simulink model "sf_aircraft_controller"  (R2025b)
settings: configuration reference "SharedConfig" (kept outside this file)
libraries: sf_aircraft_lib x4
settings Model: DataDictionary=sf_aircraft_dd.sldd  Creator=The MathWorks, Inc.  LastModifiedBy=The MathWorks, Inc.
settings ConfigSetRef: SourceName=SharedConfig

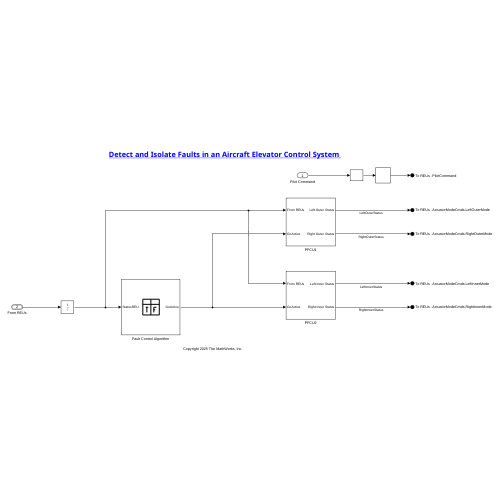
[thumbnail: Simulink's stored preview of the top-level diagram]
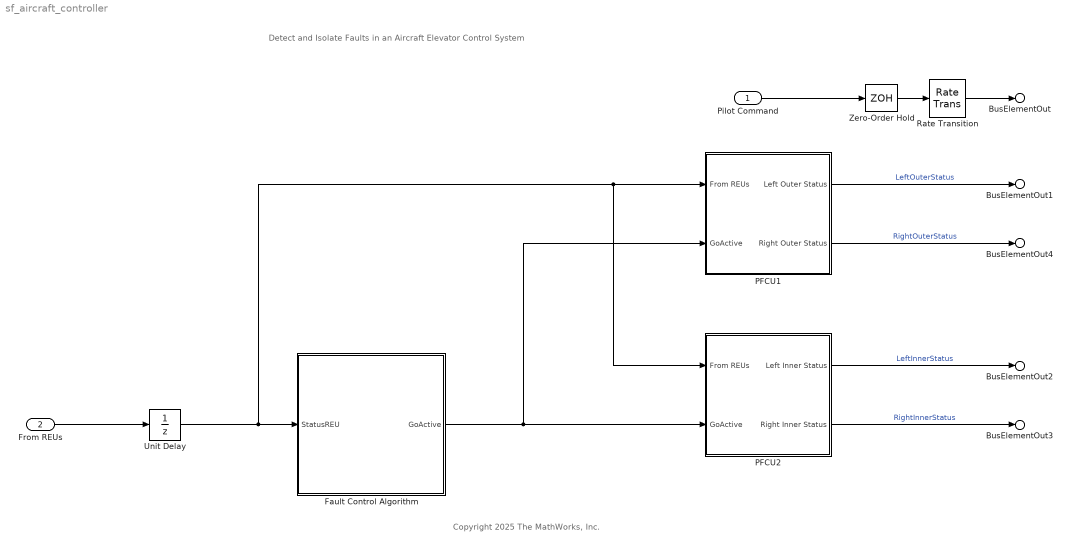
== system sf_aircraft_controller ==
  note: Copyright 2025 The MathWorks, Inc.
  note: Detect and Isolate Faults in an Aircraft Elevator Control System
  Pilot Command : Inport
  From REUs : Inport  Port=2  OutDataTypeStr=Bus: REUtoPFCU_type  PortDimensions=1  BusOutputAsStruct=on
  Fault Control Algorithm : Truth Table  TreatAsAtomicUnit=on
  PFCU1 : Subsystem
  PFCU2 : Subsystem
  Rate Transition : RateTransition  OutPortSampleTime=.01
  Unit Delay : UnitDelay  SampleTime=-1  HasFrameUpgradeWarning=on
  Zero-Order Hold : ZeroOrderHold  SampleTime=.1
  BusElementOut1 : Outport  PortName=To REUs  Element=ActuatorModeCmds.LeftOuterMode
  BusElementOut2 : Outport  PortName=To REUs  Element=ActuatorModeCmds.LeftInnerMode
  BusElementOut3 : Outport  PortName=To REUs  Element=ActuatorModeCmds.RightInnerMode
  BusElementOut4 : Outport  PortName=To REUs  Element=ActuatorModeCmds.RightOuterMode
  BusElementOut : Outport  PortName=To REUs  Element=PilotCommand
  wires:
  From REUs/1 -> Unit Delay/1
  Fault Control Algorithm/1(GoActive) -> PFCU1/2(GoActive), PFCU2/2(GoActive)
  Pilot Command/1 -> Zero-Order Hold/1
  PFCU1/1(Left Outer Status) -> BusElementOut1/1  "LeftOuterStatus"
  PFCU2/1(Left Inner Status) -> BusElementOut2/1  "LeftInnerStatus"
  PFCU2/2(Right Inner Status) -> BusElementOut3/1  "RightInnerStatus"
  PFCU1/2(Right Outer Status) -> BusElementOut4/1  "RightOuterStatus"
  Zero-Order Hold/1 -> Rate Transition/1
  Rate Transition/1 -> BusElementOut/1
  Unit Delay/1 -> PFCU1/1(From REUs), PFCU2/1(From REUs), Fault Control Algorithm/1(StatusREU)

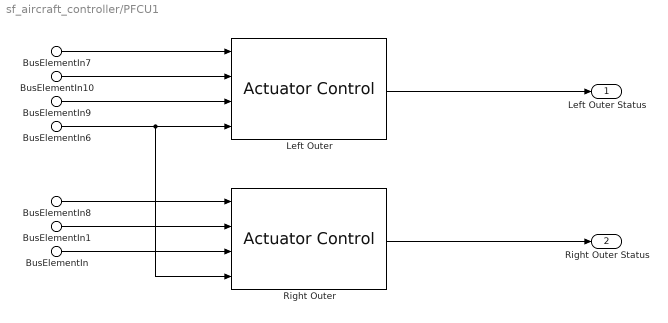
== system sf_aircraft_controller/PFCU1 ==
  BusElementIn6 : Inport  PortName=From REUs  Element=ResetCmd
  BusElementIn : Inport  PortName=From REUs  Element=RightOuterREUout.PositionFailureStatus
  BusElementIn1 : Inport  PortName=From REUs  Element=RightOuterREUout.HydraulicFailureStatus
  BusElementIn9 : Inport  PortName=From REUs  Element=LeftOuterREUout.PositionFailureStatus
  BusElementIn10 : Inport  PortName=From REUs  Element=LeftOuterREUout.HydraulicFailureStatus
  BusElementIn7 : Inport  Port=2  PortName=GoActive  Element=LeftOuterCmd
  BusElementIn8 : Inport  Port=2  PortName=GoActive  Element=RightOuterCmd
  Left Outer : sf_aircraft_lib/Actuator Control  SystemSampleTime=-1  VariantActivationTime=update diagram  EmptyChoice=off  PassThrough=off  PassThroughVariantControl=(default)  EmptyChoiceVariantControl=(default)  AllowFlexibleInterface=on  Latency=0  AutoFrameSizeCalculation=off
  Right Outer : sf_aircraft_lib/Actuator Control  SystemSampleTime=-1  VariantActivationTime=update diagram  EmptyChoice=off  PassThrough=off  PassThroughVariantControl=(default)  EmptyChoiceVariantControl=(default)  AllowFlexibleInterface=on  Latency=0  AutoFrameSizeCalculation=off
  Left Outer Status : Outport
  Right Outer Status : Outport  Port=2
  wires:
  Left Outer/1 -> Left Outer Status/1
  BusElementIn9/1 -> Left Outer/3
  BusElementIn10/1 -> Left Outer/2
  BusElementIn7/1 -> Left Outer/1
  Right Outer/1 -> Right Outer Status/1
  BusElementIn8/1 -> Right Outer/1
  BusElementIn1/1 -> Right Outer/2
  BusElementIn/1 -> Right Outer/3
  BusElementIn6/1 -> Right Outer/4, Left Outer/4

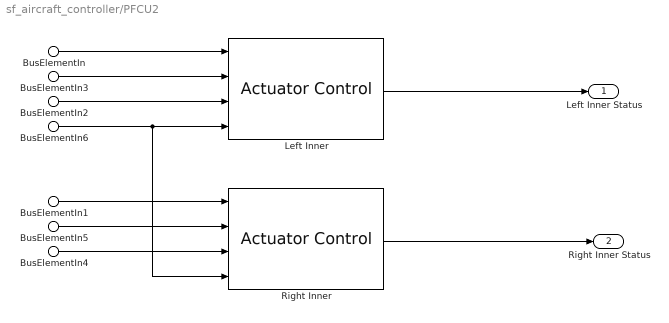
== system sf_aircraft_controller/PFCU2 ==
  BusElementIn2 : Inport  PortName=From REUs  Element=LeftInnerREUout.PositionFailureStatus
  BusElementIn3 : Inport  PortName=From REUs  Element=LeftInnerREUout.HydraulicFailureStatus
  BusElementIn4 : Inport  PortName=From REUs  Element=RightInnerREUout.PositionFailureStatus
  BusElementIn5 : Inport  PortName=From REUs  Element=RightInnerREUout.HydraulicFailureStatus
  BusElementIn6 : Inport  PortName=From REUs  Element=ResetCmd
  BusElementIn : Inport  Port=2  PortName=GoActive  Element=LeftInnerCmd
  BusElementIn1 : Inport  Port=2  PortName=GoActive  Element=RightInnerCmd
  Left Inner : sf_aircraft_lib/Actuator Control  SystemSampleTime=-1  VariantActivationTime=update diagram  EmptyChoice=off  PassThrough=off  PassThroughVariantControl=(default)  EmptyChoiceVariantControl=(default)  AllowFlexibleInterface=on  Latency=0  AutoFrameSizeCalculation=off
  Right Inner : sf_aircraft_lib/Actuator Control  SystemSampleTime=-1  VariantActivationTime=update diagram  EmptyChoice=off  PassThrough=off  PassThroughVariantControl=(default)  EmptyChoiceVariantControl=(default)  AllowFlexibleInterface=on  Latency=0  AutoFrameSizeCalculation=off
  Left Inner Status : Outport
  Right Inner Status : Outport  Port=2
  wires:
  Left Inner/1 -> Left Inner Status/1
  BusElementIn2/1 -> Left Inner/3
  BusElementIn3/1 -> Left Inner/2
  BusElementIn/1 -> Left Inner/1
  Right Inner/1 -> Right Inner Status/1
  BusElementIn1/1 -> Right Inner/1
  BusElementIn5/1 -> Right Inner/2
  BusElementIn4/1 -> Right Inner/3
  BusElementIn6/1 -> Right Inner/4, Left Inner/4

== matlab function sf_aircraft_controller/Fault Control Algorithm ==
  data: StatusREU input Bus: REUtoPFCU_type size=1; GoActive output Bus: PFCC_type
function GoActive = fcn(StatusREU)

aVarTruthTableCondition_1 = false;
aVarTruthTableCondition_2 = false;
aVarTruthTableCondition_3 = false;
aVarTruthTableCondition_4 = false;
aVarTruthTableCondition_5 = false;
aVarTruthTableCondition_6 = false;
aVarTruthTableCondition_7 = false;


% Left Outer Position || Rate

aVarTruthTableCondition_1 = logical(StatusREU.LeftOuterREUout.PositionFailureStatus);

% Hydraulic 1

aVarTruthTableCondition_2 = logical(StatusREU.LeftOuterREUout.HydraulicFailureStatus);

% Left Inner Pos || Rate

aVarTruthTableCondition_3 = logical(StatusREU.LeftInnerREUout.PositionFailureStatus);

% Hydraulic 2

aVarTruthTableCondition_4 = logical(StatusREU.LeftInnerREUout.HydraulicFailureStatus || StatusREU.RightInnerREUout.HydraulicFailureStatus);

% Right Inner Pos || Rate

aVarTruthTableCondition_5 = logical(StatusREU.RightInnerREUout.PositionFailureStatus);

% Hydraulic 3

aVarTruthTableCondition_6 = logical(StatusREU.RightOuterREUout.HydraulicFailureStatus);

% Right Outer Pos || Rate

aVarTruthTableCondition_7 = logical(StatusREU.RightOuterREUout.PositionFailureStatus);

if (~aVarTruthTableCondition_1 && ~aVarTruthTableCondition_2 && ~aVarTruthTableCondition_6 && ~aVarTruthTableCondition_7)
    aFcnTruthTableAction_1();
elseif (aVarTruthTableCondition_1 && ~aVarTruthTableCondition_3 && ~aVarTruthTableCondition_4 && ~aVarTruthTableCondition_5)
    aFcnTruthTableAction_2();
elseif (aVarTruthTableCondition_2 && ~aVarTruthTableCondition_3 && ~aVarTruthTableCondition_4 && ~aVarTruthTableCondition_5)
    aFcnTruthTableAction_2();
elseif (~aVarTruthTableCondition_3 && ~aVarTruthTableCondition_4 && ~aVarTruthTableCondition_5 && aVarTruthTableCondition_6)
    aFcnTruthTableAction_2();
elseif (~aVarTruthTableCondition_3 && ~aVarTruthTableCondition_4 && ~aVarTruthTableCondition_5 && aVarTruthTableCondition_7)
    aFcnTruthTableAction_2();
elseif (~aVarTruthTableCondition_1 && ~aVarTruthTableCondition_2 && ~aVarTruthTableCondition_5 && aVarTruthTableCondition_6)
    aFcnTruthTableAction_3();
elseif (~aVarTruthTableCondition_1 && ~aVarTruthTableCondition_2 && ~aVarTruthTableCondition_5 && aVarTruthTableCondition_7)
    aFcnTruthTableAction_3();
elseif (aVarTruthTableCondition_1 && ~aVarTruthTableCondition_3 && ~aVarTruthTableCondition_6 && ~aVarTruthTableCondition_7)
    aFcnTruthTableAction_4();
elseif (aVarTruthTableCondition_2 && ~aVarTruthTableCondition_3 && ~aVarTruthTableCondition_6 && ~aVarTruthTableCondition_7)
    aFcnTruthTableAction_4();
else % Default
    aFcnTruthTableAction_5();
end

function aFcnTruthTableAction_1()

% Left Outer + Right Outer

GoActive.LeftOuterCmd = true;
GoActive.LeftInnerCmd = false;
GoActive.RightInnerCmd = false;
GoActive.RightOuterCmd = true;

function aFcnTruthTableAction_2()

% Left Inner + Right Inner

GoActive.LeftOuterCmd = false;
GoActive.LeftInnerCmd = true;
GoActive.RightInnerCmd = true;
GoActive.RightOuterCmd = false;

function aFcnTruthTableAction_3()

% Left Outer + Right Inner

GoActive.LeftOuterCmd = true;
GoActive.LeftInnerCmd = false;
GoActive.RightInnerCmd = true;
GoActive.RightOuterCmd = false;

function aFcnTruthTableAction_4()

% Left Inner + Right Outer

GoActive.LeftOuterCmd = false;
GoActive.LeftInnerCmd = true;
GoActive.RightInnerCmd = false;
GoActive.RightOuterCmd = true;

function aFcnTruthTableAction_5()

% None

GoActive.LeftOuterCmd = false;
GoActive.LeftInnerCmd = false;
GoActive.RightInnerCmd = false;
GoActive.RightOuterCmd = false;
